simulink model "ps5_stage04_p_hardware_matched_R2024a"  (R2024a)
settings: Solver=FixedStepDiscrete  StartTime=0.0  StopTime=10  FixedStep=0.002  RelTol=1e-3
settings Model: Creator=tanuj  LastModifiedBy=tanuj

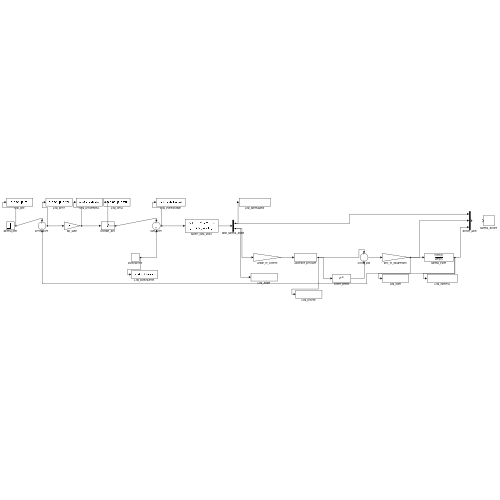
[thumbnail: Simulink's stored preview of the top-level diagram]
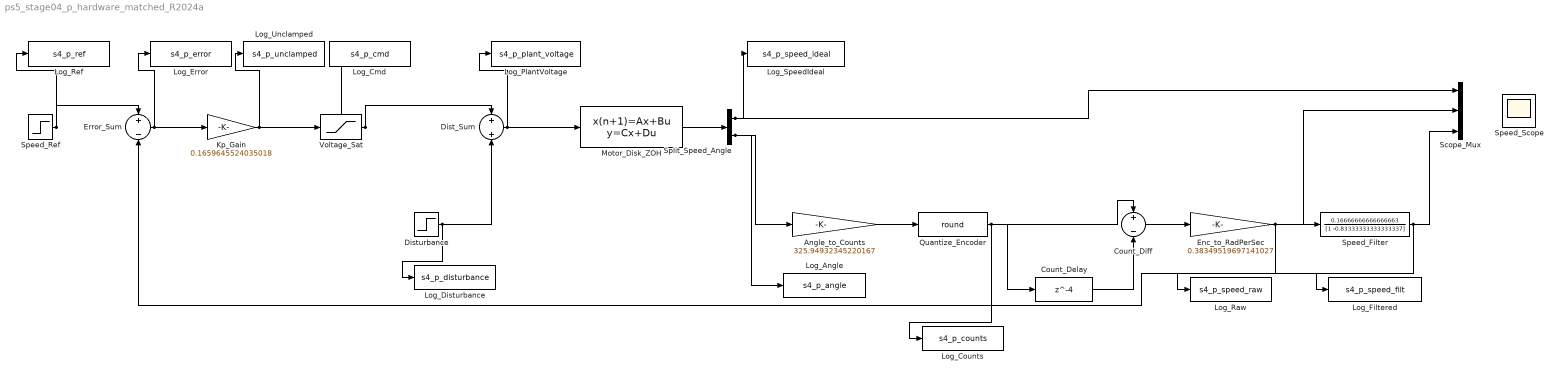
== system ps5_stage04_p_hardware_matched_R2024a ==
  Angle_to_Counts : Gain  Gain=325.94932345220167
  Count_Delay : Delay  DelayLength=4  InitialCondition=0  SampleTime=0.002
  Count_Diff : Sum  Inputs=+-
  Dist_Sum : Sum
  Disturbance : Step  Time=5  After=0.5  SampleTime=0.002
  Enc_to_RadPerSec : Gain  Gain=0.38349519697141027
  Error_Sum : Sum  Inputs=+-
  Kp_Gain : Gain  Gain=0.1659645524035018
  Log_Angle : ToWorkspace  VariableName=s4_p_angle  SampleTime=-1
  Log_Cmd : ToWorkspace  VariableName=s4_p_cmd  SampleTime=-1
  Log_Counts : ToWorkspace  VariableName=s4_p_counts  SampleTime=-1
  Log_Disturbance : ToWorkspace  VariableName=s4_p_disturbance  SampleTime=-1
  Log_Error : ToWorkspace  VariableName=s4_p_error  SampleTime=-1
  Log_Filtered : ToWorkspace  VariableName=s4_p_speed_filt  SampleTime=-1
  Log_PlantVoltage : ToWorkspace  VariableName=s4_p_plant_voltage  SampleTime=-1
  Log_Raw : ToWorkspace  VariableName=s4_p_speed_raw  SampleTime=-1
  Log_Ref : ToWorkspace  VariableName=s4_p_ref  SampleTime=-1
  Log_SpeedIdeal : ToWorkspace  VariableName=s4_p_speed_ideal  SampleTime=-1
  Log_Unclamped : ToWorkspace  VariableName=s4_p_unclamped  SampleTime=-1
  Motor_Disk_ZOH : DiscreteStateSpace  A=[-0.0019480304943638347 -0.0055041701060564701 0;0.34591769089835145 0.9762812537573784 0;0.00064636393789134212 0.0019778638926502613 1]  B=[0.13043057123356561;0.56205559816638462;0.00052455230686583696]  C=[0 1 0;0 0 1]  D=[0;0]  SampleTime=0.002
  Quantize_Encoder : Rounding  Operator=round
  Scope_Mux : Mux  Inputs=3
  Speed_Filter : DiscreteFilter  Numerator=0.16666666666666663  Denominator=[1 -0.83333333333333337]  SampleTime=0.002
  Speed_Ref : Step  After=50  SampleTime=0.002
  Speed_Scope : Scope
  Split_Speed_Angle : Demux  Outputs=2
  Voltage_Sat : Saturate  UpperLimit=10  LowerLimit=-10
  wires:
  Speed_Ref/1 -> Error_Sum/1, Log_Ref/1
  Error_Sum/1 -> Kp_Gain/1, Log_Error/1
  Kp_Gain/1 -> Voltage_Sat/1, Log_Unclamped/1
  Voltage_Sat/1 -> Dist_Sum/1, Log_Cmd/1
  Disturbance/1 -> Dist_Sum/2, Log_Disturbance/1
  Dist_Sum/1 -> Motor_Disk_ZOH/1, Log_PlantVoltage/1
  Motor_Disk_ZOH/1 -> Split_Speed_Angle/1
  Split_Speed_Angle/2 -> Angle_to_Counts/1, Log_Angle/1
  Angle_to_Counts/1 -> Quantize_Encoder/1
  Quantize_Encoder/1 -> Count_Diff/1, Count_Delay/1, Log_Counts/1
  Count_Delay/1 -> Count_Diff/2
  Count_Diff/1 -> Enc_to_RadPerSec/1
  Enc_to_RadPerSec/1 -> Speed_Filter/1, Log_Raw/1, Scope_Mux/2
  Speed_Filter/1 -> Error_Sum/2, Log_Filtered/1, Scope_Mux/3
  Split_Speed_Angle/1 -> Log_SpeedIdeal/1, Scope_Mux/1
